simulink model "q2s"  (R2022a)
settings: Solver=VariableStepAuto  StartTime=0.0  StopTime=10.0  RelTol=1e-3
settings Model: Creator=giova  LastModifiedBy=giova

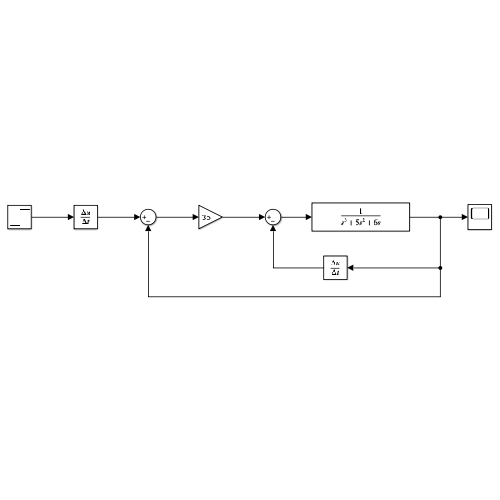
[thumbnail: Simulink's stored preview of the top-level diagram]
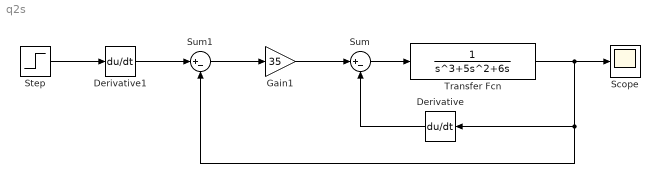
== system q2s ==
  Derivative : Derivative
  Derivative1 : Derivative
  Gain1 : Gain  Gain=35
  Scope : Scope
  Step : Step  SampleTime=0
  Sum : Sum  Inputs=|+-
  Sum1 : Sum  Inputs=|+-
  Transfer Fcn : TransferFcn  Denominator=[1 5 6 0]
  wires:
  Sum1/1 -> Gain1/1
  Gain1/1 -> Sum/1
  Sum/1 -> Transfer Fcn/1
  Transfer Fcn/1 -> Derivative/1, Sum1/2, Scope/1
  Step/1 -> Derivative1/1
  Derivative1/1 -> Sum1/1
  Derivative/1 -> Sum/2
